simulink model "sm_car_"  (R2026b)
settings: Solver=ode23t  StopTime=100  MaxStep=0.4  AbsTol=1e-3  EnableMultiTasking=on
PreLoadFcn:
  | % Due to usability issue in Repeating Sequence block
  | warning('off','Simulink:Masking:Invalid');
  | 
  | % Eliminate unnecessary warnings in inactive variants
  | % Warnings generated only if you click through inactive variant
  | warning('off','MATLAB:nonExistentField');
  | warning('off','Simulink:Parameters:BlkParamUndefined');
PostLoadFcn:
  | set_param([bdroot '/Vehicle'],'popup_trailer','Off')
  | warning('off','sm:sli:setup:compile:LocalSolverNotSupported')
  | %sm_car_config_maneuver(bdroot,'WOT Braking');
  | sm_car_config_vehicle(bdroot,'false');
  | sm_car_config_logging(bdroot);
InitFcn:
  | sm_car_config_camera;
  | Vehicle = sm_car_vehcfg_checkConfig(Vehicle);
  | sm_car_check_tire_model(bdroot);
StartFcn:
  | tic;
StopFcn:
  | Elapsed_Sim_Time = toc;
  | % disp(['Elapsed Sim Time = ' num2str(Elapsed_Sim_Time)]);
undefined symbols (not defined in the file or in its folder): acc_theta, accel_ramp_rate, Axle1D, AxleIn, Camera, Control, Driver, Init, Maneuver, Pedal, Scene, ShaftL1, ShaftL2, ShaftR1, ShaftR2, Visual, X, xy_data_car_side, Y, Z
libraries: sm_lib x290, fl_lib x171, nesl_utility x144, simulink x60, simulink_extras x14, sdl_lib x14, SimscapeFluids_lib x7, Damper_Element x4, Tire_1x2x x4, ee_lib x3, Scene_Utilities x3, sharedTrackingLibrary x2
(part 1 of 22)
CloseFcn:
  | try,close(h1_sm_car),end
  | clear h1_sm_car
  | try,close(h2_sm_car),end
  | clear h2_sm_car
  | try,close(h3_sm_car),end
  | clear h3_sm_car
  | try,close(h4_sm_car),end
  | clear h4_sm_car
  | 
  | 
  | clear simlog_sm_car
  | clear logsout_sm_car
settings Model: SimulationMode=accelerator  Creator=smiller  LastModifiedBy=andrei
settings SolverCC: AutoInsertRateTranBlk=on  InsertRTBMode=Never (minimum delay)  MaxConsecutiveMinStep=5  MinimalZcImpactIntegration=on
settings DataIOCC: DSMLogging=off  MaxDataPoints=10000  ReturnWorkspaceOutputs=off  SaveFormat=StructureWithTime  SaveOutput=off  SignalLoggingName=logsout_sm_car
settings OptimizationCC: BlockReduction=off  BufferReuse=off  BusAssignmentInplaceUpdate=off  ExpressionFolding=off  GlobalBufferReuse=off  LocalBlockOutputs=off  OptimizeBlockIOStorage=off  OptimizeDataStoreBuffers=off  ReuseModelBlockBuffer=off  UseDivisionForNetSlopeComputation=on
settings DebuggingCC: AlgebraicLoopMsg=none  ArithmeticOperatorsInVariantConditions=warning  ParameterPrecisionLossMsg=none
settings HardwareCC: ProdHWDeviceType=Generic->32-bit x86 compatible  ProdLargestAtomicFloat=None  ProdLongLongMode=on
settings SFSimCC: CustomCodeUndefinedFunction=UseInterfaceOnly
settings RTWCC: DLArmComputeVersion=19.05
settings GRTTargetCC: TargetLangStandard=C89/C90 (ANSI)
settings SimscapeCC: SimscapeLogName=simlog_sm_car  SimscapeLogSimulationStatistics=on  SimscapeLogType=all  SimscapeOperatingPoint=ssc_op  SimscapeUseEnergyAccounting=off
settings DiagnosticsConfigSet: SimMechanicsConflictingReferenceFrames=none  SimMechanicsRigidlyBoundBlock=none  SimMechanicsUnsatisfiedHighPriorityTargets=error
settings ExplorerConfigSet: InternalSimMechanicsExplorerSettings="<ExplorerConfiguration><canonicalview>default</canonicalview><AnimationSetting><BasePlaybackSpeed>1.0</BasePlaybackSpeed><PlaybackSpeedFactor>1.0</PlaybackSpeedFactor></AnimationSetting><TilePanel><TileInfo><Tiles Columns=\"1\" Count=\"1\" Rows=\"1\"><Column Weight=\"1\"/><Row Weight=\"1\"/><Tile Height=\"1\" Width=\"1\" X=\"0\" Y=\"0\"/></Tiles></TileInfo><SceneInfo><SceneViewer><BGColor><R>1</R><G>1</G><B>1</B></BGColor><Camera><DoPerspective>on</DoPerspective><Position><X>-22.5734563329168161</X><Y>-2.56079992530625722</Y><Z>1.4393604008155032</Z></Position><Center><X>-23.2962680852000119</X><Y>-1.95845679840359432</Y><Z>1.10064823948317181</Z></Center><Up><X>-0.260205889993916473</X><Y>0.216838241661597014</Y><Z>0.940890042335224552</Z></Up><ViewLimDist>1</ViewLimDist><YLim>0.466307658154998694</YLim><XLim>0.489818968650208741</XLim></Camera></SceneViewer></SceneInfo></TilePanel><MechEditorPanel><Cameras><Camera><Id>Camera1</Id><Value><Name>Track FixO FR</Name><NativeCamera><PositionTrackingFeature>Camera_Frames.Frame_FixO_FR.R</PositionTrackingFeature><CenterTrackingFeature>Camera_Frames.Frame_FixO_FR.R</CenterTrackingFeature><UpVectorTrackingFeature>Camera_Frames.Frame_FixO_FR.R</UpVectorTrackingFeature><CenterTrackingOrigin>off</CenterTrackingOrigin><CenterTrackingDirection>+X</CenterTrackingDirection><UpVectorTrackingDirection>+Z</UpVectorTrackingDirection></NativeCamera></Value></Camera><Camera><Id>Camera2</Id><Value><Name>Track FixO Right</Name><NativeCamera><PositionTrackingFeature>Camera_Frames.Frame_FixO_Right.R</PositionTrackingFeature><CenterTrackingFeature>Camera_Frames.Transform_Camera_Ref.F</CenterTrackingFeature><UpVectorTrackingFeature>Camera_Frames.Frame_FixO_Right.R</UpVectorTrackingFeature><CenterTrackingOrigin>off</CenterTrackingOrigin><CenterTrackingDirection>+Y</CenterTrackingDirection><UpVectorTrackingDirection>+Z</UpVectorTrackingDirection></NativeCamera></Value></Camera><Camera><Id>Camera3</Id><Value><Name>Track FixO RR</Name><NativeCamera><PositionTrackingFeature>Camera_Frames.Frame_FixO_RR.R</PositionTrackingFeature><CenterTrackingFeature>Camera_Frames.Frame_FixO_RR.R</CenterTrackingFeature><UpVectorTrackingFeature>Camera_Frames.Frame_FixO_RR.R</UpVectorTrackingFeature><CenterTrackingOrigin>off</CenterTrackingOrigin><CenterTrackingDirection>+X</CenterTrackingDirection><UpVectorTrackingDirection>+Z</UpVectorTrackingDirection></NativeCamera></Value></Camera><Camera><Id>Camera4</Id><Value><Name>Track FixO RL</Name><NativeCamera><PositionTrackingFeature>Camera_Frames.Frame_FixO_RL.R</PositionTrackingFeature><CenterTrackingFeature>Camera_Frames.Frame_FixO_RL.R</CenterTrackingFeature><UpVectorTrackingFeature>Camera_Frames.Frame_FixO_RL.R</UpVectorTrackingFeature><CenterTrackingOrigin>off</CenterTrackingOrigin><CenterTrackingDirection>+X</CenterTrackingDirection><UpVectorTrackingDirection>+Z</UpVectorTrackingDirection></NativeCamera></Value></Camera><Camera><Id>Camera5</Id><Value><Name>Track FixO Left</Name><NativeCamera><PositionTrackingFeature>Camera_Frames.Frame_FixO_Left.R</PositionTrackingFeature><CenterTrackingFeature>Camera_Frames.Transform_Camera_Ref.F</CenterTrackingFeature><UpVectorTrackingFeature>Camera_Frames.Frame_FixO_Left.R</UpVectorTrackingFeature><CenterTrackingOrigin>off</CenterTrackingOrigin><CenterTrackingDirection>-Y</CenterTrackingDirection><UpVectorTrackingDirection>+Z</UpVectorTrackingDirection></NativeCamera></Value></Camera><Camera><Id>Camera6</Id><Value><Name>Track FixO FL</Name><NativeCamera><PositionTrackingFeature>Camera_Frames.Frame_FixO_FL.R</PositionTrackingFeature><CenterTrackingFeature>Camera_Frames.Frame_FixO_FL.R</CenterTrackingFeature><UpVectorTrackingFeature>Camera_Frames.Frame_FixO_FL.R</UpVectorTrackingFeature><CenterTrackingOrigin>off</CenterTrackingOrigin><CenterTrackingDirection>+X</CenterTrackingDirection><UpVectorTrackingDirection>+Z</UpVectorTrackingDirection></NativeCamera></Value></Camera><Camera><Id>Camera7</Id><Value><Name>Track FixO Top</Name><NativeCamera><PositionTrackingFeature>Camera_Frames.Frame_FixO_Top.R</PositionTrackingFeature><CenterTrackingFeature>Camera_Frames.Frame_FixO_Top.R</CenterTrackingFeature><UpVectorTrackingFeature>Camera_Frames.Frame_FixO_Top.R</UpVectorTrackingFeature><CenterTrackingOrigin>off</CenterTrackingOrigin><CenterTrackingDirection>+X</CenterTrackingDirection><UpVectorTrackingDirection>+Z</UpVectorTrackingDirection></NativeCamera></Value></Camera><Camera><Id>Camera8</Id><Value><Name>Track FixO Front</Name><NativeCamera><PositionTrackingFeature>Camera_Frames.Frame_FixO_Front.R</PositionTrackingFeature><CenterTrackingFeature>Camera_Frames.Frame_FixO_Front.R</CenterTrackingFeature><UpVectorTrackingFeature>Camera_Frames.Frame_FixO_Front.R</UpVectorTrackingFeature><CenterTrackingOrigin>off</CenterTrackingOrigin><CenterTrackingDirection>+X</CenterTrackingDirection><UpVectorTrackingDirection>+Z</UpVectorTrackingDirection></NativeCamera></Value></Camera><Camera><Id>Camera9</Id><Value><Name>Track FixO Rear</Name><NativeCamera><PositionTrackingFeature>Camera_Frames.Frame_FixO_Rear.R</PositionTrackingFeature><CenterTrackingFeature>Camera_Frames.Frame_FixO_Rear.R</CenterTrackingFeature><UpVectorTrackingFeature>Camera_Frames.Frame_FixO_Rear.R</UpVectorTrackingFeature><CenterTrackingOrigin>off</CenterTrackingOrigin><CenterTrackingDirection>+X</CenterTrackingDirection><UpVectorTrackingDirection>+Z</UpVectorTrackingDirection></NativeCamera></Value></Camera><Camera><Id>Camera10</Id><Value><Name>Track FR</Name><NativeCamera><PositionTrackingFeature>Camera_Frames.Frame_FR.R</PositionTrackingFeature><CenterTrackingFeature>Camera_Frames.Frame_FR.R</CenterTrackingFeature><UpVectorTrackingFeature>Camera_Frames.Frame_FR.R</UpVectorTrackingFeature><CenterTrackingOrigin>off</CenterTrackingOrigin><CenterTrackingDirection>+X</CenterTrackingDirection><UpVectorTrackingDirection>+Z</UpVectorTrackingDirection></NativeCamera></Value></Camera><Camera><Id>Camera11</Id><Value><Name>Track Right</Name><NativeCamera><PositionTrackingFeature>Camera_Frames.Frame_Right.R</PositionTrackingFeature><CenterTrackingFeature>Camera_Frames.Transform_Camera_Ref.F</CenterTrackingFeature><UpVectorTrackingFeature>Camera_Frames.Frame_Right.R</UpVectorTrackingFeature><CenterTrackingOrigin>off</CenterTrackingOrigin><CenterTrackingDirection>+Y</CenterTrackingDirection><UpVectorTrackingDirection>+Z</UpVectorTrackingDirection></NativeCamera></Value></Camera><Camera><Id>Camera12</Id><Value><Name>Track RR</Name><NativeCamera><PositionTrackingFeature>Camera_Frames.Frame_RR.R</PositionTrackingFeature><CenterTrackingFeature>Camera_Frames.Frame_RR.R</CenterTrackingFeature><UpVectorTrackingFeature>Camera_Frames.Frame_RR.R</UpVectorTrackingFeature><CenterTrackingOrigin>off</CenterTrackingOrigin><CenterTrackingDirection>+X</CenterTrackingDirection><UpVectorTrackingDirection>+Z</UpVectorTrackingDirection></NativeCamera></Value></Camera><Camera><Id>Camera13</Id><Value><Name>Track RL</Name><NativeCamera><PositionTrackingFeature>Camera_Frames.Frame_RL.R</PositionTrackingFeature><CenterTrackingFeature>Camera_Frames.Frame_RL.R</CenterTrackingFeature><UpVectorTrackingFeature>Camera_Frames.Frame_RL.R</UpVectorTrackingFeature><CenterTrackingOrigin>off</CenterTrackingOrigin><CenterTrackingDirection>+X</CenterTrackingDirection><UpVectorTrackingDirection>+Z</UpVectorTrackingDirection></NativeCamera></Value></Camera><Camera><Id>Camera14</Id><Value><Name>Track Left</Name><NativeCamera><PositionTrackingFeature>Camera_Frames.Frame_Left.R</PositionTrackingFeature><CenterTrackingFeature>Camera_Frames.Transform_Camera_Ref.F</CenterTrackingFeature><UpVectorTrackingFeature>Camera_Frames.Frame_Left.R</UpVectorTrackingFeature><CenterTrackingOrigin>off</CenterTrackingOrigin><CenterTrackingDirection>-Y</CenterTrackingDirection><UpVectorTrackingDirection>+Z</UpVectorTrackingDirection></NativeCamera></Value></Camera><Camera><Id>Camera15</Id><Value><Name>Track FL</Name><NativeCamera><PositionTrackingFeature>Camera_Frames.Frame_FL.R</PositionTrackingFeature><CenterTrackingFeature>Camera_Frames.Frame_FL.R</CenterTrackingFeature><UpVectorTrackingFeature>Camera_Frames.Frame_FL.R</UpVectorTrackingFeature><CenterTrackingOrigin>off</CenterTrackingOrigin><CenterTrackingDirection>+X</CenterTrackingDirection><UpVectorTrackingDirection>+Z</UpVectorTrackingDirection></NativeCamera></Value></Camera><Camera><Id>Camera16</Id><Value><Name>Track Top</Name><NativeCamera><PositionTrackingFeature>Camera_Frames.Frame_Top.R</PositionTrackingFeature><CenterTrackingFeature>Camera_Frames.Frame_Top.R</CenterTrackingFeature><UpVectorTrackingFeature>Camera_Frames.Frame_Top.R</UpVectorTrackingFeature><CenterTrackingOrigin>off</CenterTrackingOrigin><CenterTrackingDirection>+X</CenterTrackingDirection><UpVectorTrackingDirection>+Z</UpVectorTrackingDirection></NativeCamera></Value></Camera><Camera><Id>Camera17</Id><Value><Name>Track Front</Name><NativeCamera><PositionTrackingFeature>Camera_Frames.Frame_Front.R</PositionTrackingFeature><CenterTrackingFeature>Camera_Frames.Frame_Front.R</CenterTrackingFeature><UpVectorTrackingFeature>Camera_Frames.Frame_Front.R</UpVectorTrackingFeature><CenterTrackingOrigin>off</CenterTrackingOrigin><CenterTrackingDirection>+X</CenterTrackingDirection><UpVectorTrackingDirection>+Z</UpVectorTrackingDirection></NativeCamera></Value></Camera><Camera><Id>Camera18</Id><Value><Name>Track Rear</Name><NativeCamera><PositionTrackingFeature>Camera_Frames.Frame_Rear.R</PositionTrackingFeature><CenterTrackingFeature>Camera_Frames.Frame_Rear.R</CenterTrackingFeature><UpVectorTrackingFeature>Camera_Frames.Frame_Rear.R</UpVectorTrackingFeature><CenterTrackingOrigin>off</CenterTrackingOrigin><CenterTrackingDirection>+X</CenterTrackingDirection><UpVectorTrackingDirection>+Z</UpVectorTrackingDirection></NativeCamera></Value></Camera><Camera><Id>Camera19</Id><Value><Name>Track SuspF</Name><NativeCamera><PositionTrackingFeature>Camera_Frames.Frame_SuspF.R</PositionTrackingFeature><CenterTrackingFeature>Camera_Frames.Frame_SuspF.R</CenterTrackingFeature><UpVectorTrackingFeature>Camera_Frames.Frame_SuspF.R</UpVectorTrackingFeature><CenterTrackingOrigin>off</CenterTrackingOrigin><CenterTrackingDirection>+X</CenterTrackingDirection><UpVectorTrackingDirection>+Z</UpVectorTrackingDirection></NativeCamera></Value></Camera><Camera><Id>Camera20</Id><Value><Name>Track SuspR</Name><NativeCamera><PositionTrackingFeature>Camera_Frames.Frame_SuspR.R</PositionTrackingFeature><CenterTrackingFeature>Camera_Frames.Frame_SuspR.R</CenterTrackingFeature><UpVectorTrackingFeature>Camera_Frames.Frame_SuspR.R</UpVectorTrackingFeature><CenterTrackingOrigin>off</CenterTrackingOrigin><CenterTrackingDirection>+X</CenterTrackingDirection><UpVectorTrackingDirection>+Z</UpVectorTrackingDirection></NativeCamera></Value></Camera><Camera><Id>Camera21</Id><Value><Name>Track WheelFR</Name><NativeCamera><PositionTrackingFeature>Camera_Frames.Frame_Wheel_FR.R</PositionTrackingFeature><CenterTrackingFeature>Camera_Frames.Frame_Wheel_FR.R</CenterTrackingFeature><UpVectorTrackingFeature>Camera_Frames.Frame_Wheel_FR.R</UpVectorTrackingFeature><CenterTrackingOrigin>off</CenterTrackingOrigin><CenterTrackingDirection>+X</CenterTrackingDirection><UpVectorTrackingDirection>+Z</UpVectorTrackingDirection></NativeCamera></Value></Camera><Camera><Id>Camera22</Id><Value><Name>Track WheelRR</Name><NativeCamera><PositionTrackingFeature>Camera_Frames.Frame_Wheel_RR.R</PositionTrackingFeature><CenterTrackingFeature>Camera_Frames.Frame_Wheel_RR.R</CenterTrackingFeature><UpVectorTrackingFeature>Camera_Frames.Frame_Wheel_RR.R</UpVectorTrackingFeature><CenterTrackingOrigin>off</CenterTrackingOrigin><CenterTrackingDirection>+X</CenterTrackingDirection><UpVectorTrackingDirection>+Z</UpVectorTrackingDirection></NativeCamera></Value></Camera><Camera><Id>Camera23</Id><Value><Name>Track WheelRL</Name><NativeCamera><PositionTrackingFeature>Camera_Frames.Frame_Wheel_RL.R</PositionTrackingFeature><CenterTrackingFeature>Camera_Frames.Frame_Wheel_RL.R</CenterTrackingFeature><UpVectorTrackingFeature>Camera_Frames.Frame_Wheel_RL.R</UpVectorTrackingFeature><CenterTrackingOrigin>off</CenterTrackingOrigin><CenterTrackingDirection>+X</CenterTrackingDirection><UpVectorTrackingDirection>+Z</UpVectorTrackingDirection></NativeCamera></Value></Camera><Camera><Id>Camera24</Id><Value><Name>Track WheelFL</Name><NativeCamera><PositionTrackingFeature>Camera_Frames.Frame_Wheel_FL.R</PositionTrackingFeature><CenterTrackingFeature>Camera_Frames.Frame_Wheel_FL.R</CenterTrackingFeature><UpVectorTrackingFeature>Camera_Frames.Frame_Wheel_FL.R</UpVectorTrackingFeature><CenterTrackingOrigin>off</CenterTrackingOrigin><CenterTrackingDirection>+X</CenterTrackingDirection><UpVectorTrackingDirection>+Z</UpVectorTrackingDirection></NativeCamera></Value></Camera><Camera><Id>Camera25</Id><Value><Name>View Seat FL</Name><NativeCamera><PositionTrackingFeature>Camera_Frames.Frame_View_Seat_FL.R</PositionTrackingFeature><CenterTrackingFeature>Camera_Frames.Frame_View_Seat_FL.R</CenterTrackingFeature><UpVectorTrackingFeature>Camera_Frames.Frame_View_Seat_FL.R</UpVectorTrackingFeature><CenterTrackingOrigin>off</CenterTrackingOrigin><CenterTrackingDirection>+X</CenterTrackingDirection><UpVectorTrackingDirection>+Z</UpVectorTrackingDirection></NativeCamera></Value></Camera><Camera><Id>Camera26</Id><Value><Name>View Seat FR</Name><NativeCamera><PositionTrackingFeature>Camera_Frames.Frame_View_Seat_FR.R</PositionTrackingFeature><CenterTrackingFeature>Camera_Frames.Frame_View_Seat_FR.R</CenterTrackingFeature><UpVectorTrackingFeature>Camera_Frames.Frame_View_Seat_FR.R</UpVectorTrackingFeature><CenterTrackingOrigin>off</CenterTrackingOrigin><CenterTrackingDirection>+X</CenterTrackingDirection><UpVectorTrackingDirection>+Z</UpVectorTrackingDirection></NativeCamera></Value></Camera><Camera><Id>Camera27</Id><Value><Name>View Susp FR</Name><NativeCamera><PositionTrackingFeature>Camera_Frames.Frame_View_Susp_FR.R</PositionTrackingFeature><CenterTrackingFeature>Camera_Frames.Frame_View_Susp_FR.R</CenterTrackingFeature><UpVectorTrackingFeature>Camera_Frames.Frame_View_Susp_FR.R</UpVectorTrackingFeature><CenterTrackingOrigin>off</CenterTrackingOrigin><CenterTrackingDirection>+X</CenterTrackingDirection><UpVectorTrackingDirection>+Z</UpVectorTrackingDirection></NativeCamera></Value></Camera><Camera><Id>Camera28</Id><Value><Name>View Susp RR</Name><NativeCamera><PositionTrackingFeature>Camera_Frames.Frame_View_Susp_RR.R</PositionTrackingFeature><CenterTrackingFeature>Camera_Frames.Frame_View_Susp_RR.R</CenterTrackingFeature><UpVectorTrackingFeature>Camera_Frames.Frame_View_Susp_RR.R</UpVectorTrackingFeature><CenterTrackingOrigin>off</CenterTrackingOrigin><CenterTrackingDirection>+X</CenterTrackingDirection><UpVectorTrackingDirection>+Z</UpVectorTrackingDirection></NativeCamera></Value></Camera><Camera><Id>Camera29</Id><Value><Name>View Susp RL</Name><NativeCamera><PositionTrackingFeature>Camera_Frames.Frame_View_Susp_RL.R</PositionTrackingFeature><CenterTrackingFeature>Camera_Frames.Frame_View_Susp_RL.R</CenterTrackingFeature><UpVectorTrackingFeature>Camera_Frames.Frame_View_Susp_RL.R</UpVectorTrackingFeature><CenterTrackingOrigin>off</CenterTrackingOrigin><CenterTrackingDirection>+X</CenterTrackingDirection><UpVectorTrackingDirection>+Z</UpVectorTrackingDirection></NativeCamera></Value></Camera><Camera><Id>Camera30</Id><Value><Name>View Susp FL</Name><NativeCamera><PositionTrackingFeature>Camera_Frames.Frame_View_Susp_FL.R</PositionTrackingFeature><CenterTrackingFeature>Camera_Frames.Frame_View_Susp_FL.R</CenterTrackingFeature><UpVectorTrackingFeature>Camera_Frames.Frame_View_Susp_FL.R</UpVectorTrackingFeature><CenterTrackingOrigin>off</CenterTrackingOrigin><CenterTrackingDirection>+X</CenterTrackingDirection><UpVectorTrackingDirection>+Z</UpVectorTrackingDirection></NativeCamera></Value></Camera><Camera><Id>Camera31</Id><Value><Name>Dolly Camera</Name><NativeCamera><PositionTrackingFeature>Camera_Frames.Frame_Dolly.R</PositionTrackingFeature><CenterTrackingFeature>Camera_Frames.Frame_Dolly.R</CenterTrackingFeature><UpVectorTrackingFeature>Camera_Frames.Frame_Dolly.R</UpVectorTrackingFeature><CenterTrackingOrigin>off</CenterTrackingOrigin><CenterTrackingDirection>+X</CenterTrackingDirection><UpVectorTrackingDirection>+Z</UpVectorTrackingDirection></NativeCamera></Value></Camera><Camera><Id>Camera32</Id><Value><Name>Track Dolly Camera</Name><NativeCamera><PositionTrackingFeature>Camera_Frames.Frame_Dolly.R</PositionTrackingFeature><CenterTrackingFeature>Camera_Frames.Transform_Camera_Ref.F</CenterTrackingFeature><UpVectorTrackingFeature>Camera_Frames.World_Frame.W</UpVectorTrackingFeature><CenterTrackingOrigin>on</CenterTrackingOrigin><UpVectorTrackingDirection>+Z</UpVectorTrackingDirection></NativeCamera></Value></Camera></Cameras><GfxPanelCameraMap><MapElement CameraMLId=\"Camera1\" GfxPanelIndex=\"0\"/></GfxPanelCameraMap><VideoCreator><PlaybackSpeedRatio>1.0</PlaybackSpeedRatio><FrameRate>30</FrameRate><VideoFormat>MPEG-4</VideoFormat><FrameSize>[800 450]</FrameSize></VideoCreator></MechEditorPanel></ExplorerConfiguration>"

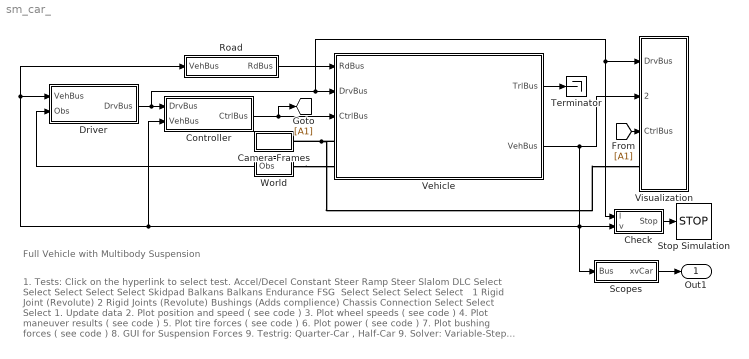
== system sm_car_ ==
  note: Full Vehicle with Multibody Suspension
  note: 1. Tests: Click on the hyperlink to select test.
      | Accel/Decel
      | Constant Steer
      | Ramp Steer
      | Slalom
      | DLC
      |
      | Select
      | Select
      | Select
      | Select
      | Select
      |
      | Skidpad
      | Balkans
      | Balkans Endurance
      | FSG
      | ​
      |
      | Select
      | Select
      | Select
      | Select
      | ​
      |
      | ​
      | 1 Rigid Joint
      | (Revolute)
      | 2 Rigid Joints
      | (Revolute)
      | Bushings
      | (Adds complience)
      |
      | Chassis Connection
      | Select
      | Select
      | Select
      |
      | 1. Update data
      | 2. Plot position and speed ( see code )
      | 3. Plot wheel speeds ( see code )
      | 4. Plot maneuver results ( see code )
      | 5. Plot tire forces ( see code )
      | 6. Plot power ( see code )
      | 7. Plot bushing forces ( see code )
      | 8. GUI for Suspension Forces
      | 9. Testrig: Quarter-Car , Half-Car
      |
      | 9. Solver: Variable-Step , Fixed Step ( see code )
      | 10. Explore simulation results using sscexplore
      | 11. Learn more about this model.
  Camera Frames : Subsystem  mask(Camera Frame Definitions){Camera=Camera, popup_dolly_camera=Off}
      mask prompts: popup_dolly_camera "Dolly Camera"
      mask help: Defines set of camera frames surrounding vehicle. Frames are used to define visualization viewpoints for animation of simulation results.
      mask init:
      | set_param([gcb '/Dolly Camera'],'LabelModeActiveChoice',get_param(gcb,'popup_dolly_camera'));
      mask TypeOptions popup_dolly_camera: Off | XYZ
      mask Display: disp('Cam')
  Check : Subsystem  mask(Stop Conditions){stop_speed=0.1, start_check_time=5, max_speed=0.4, start_check_time_max_speed=20000, lat_dev_threshold=4, start_check_time_ld=4, End_Lap=0.2, start_check_end_lap=20000, Final_lap=1, Time_Lap_Final=10000, max_dist_threshold=Maneuver.xMax.Value, start_check_time_max_dist=2}
      mask help: Check conditions of vehicle to determine if simulation should stop. Conditions can include speed, position, or end of lap. Set time to start check to very high values to prevent condition from stopping simulation.
      mask TypeOptions stop_speed: Stop Threshold/Value
      mask TypeOptions start_check_time: Start Checking/Time
      mask TypeOptions max_speed: Max Speed Threshold/Value
      mask TypeOptions start_check_time_max_speed: Start Checking Max Speed/Time
      mask TypeOptions lat_dev_threshold: Lateral Deviation Threshold/Value
      mask TypeOptions start_check_time_ld: Start Checking Lat Dev/Time
      mask TypeOptions End_Lap: End Lap/Value
      mask TypeOptions start_check_end_lap: Start Checking End Lap/Time
      mask TypeOptions Final_lap: End Laps/Value
      mask TypeOptions Time_Lap_Final: Start Checking Final Lap/Time
      mask TypeOptions max_dist_threshold: End Distance/Value
      mask TypeOptions start_check_time_max_dist: Start Checking End Distance/Time
      mask DialogControl text_quantity Prompt: Quantity
      mask DialogControl text_start_check Prompt: Start Check (sec)
      mask DialogControl text_final_speed Prompt: Final Speed (m/s)
      mask DialogControl text_max_speed Prompt: Max Speed (m/s)
      mask DialogControl text_max_lat_dev Prompt: Max Lateral Offset (m)
      mask DialogControl text_end_lap Prompt: End Lap
      mask DialogControl text_final_lap Prompt: Final Lap
      mask DialogControl text_max_distance Prompt: Max Distance
  Controller : Subsystem  Variant=on  VariantControlMode=label  VariantControl=Variant1  LabelModeActiveChoice=Default  mask(Control){popup_control=Default, popup_brake_control=Pedal}
      mask prompts: popup_control "Control"; popup_brake_control "Brake Control"
      mask help: Models vehicle controller behavior. Takes commands from driver and produces inputs for vehicle systems including braking, steering, and powertrain.
      mask init:
      | temp_ctrlMode = get_param(gcb,'popup_control');
      | if(strcmp(temp_ctrlMode,'Default'))
      |     set_param(gcb,'LabelModeActiveChoice','Default');
      |     set_param([gcb '/Default'],'popup_brake_control',...
      |         get_param(gcb,'popup_brake_control'))
      | elseif(strcmp(temp_ctrlMode,'Fuel Cell 1 Motor'))
      |     set_param(gcb,'LabelModeActiveChoice','FuelCell1Motor');
      | elseif(strcmp(temp_ctrlMode,'Battery 2 Motor'))
      |     set_param(gcb,'LabelModeActiveChoice','Battery2Motor');
      | elseif(strcmp(temp_ctrlMode,'Torque Vector 4 Motor'))
      |     set_param(gcb,'LabelModeActiveChoice','TrqVec_4Motor');
      |     set_param([gcb '/TrqVec 4Motor'],'popup_brake_control',...
      |         get_param(gcb,'popup_brake_control'))
      | elseif(strcmp(temp_ctrlMode,'TrqVecARTTU'))
      |         set_param(gcb,'LabelModeActiveChoice','TrqVecARTTU');
      | elseif(strcmp(temp_ctrlMode,'FLC_DYC'))
      |         set_param(gcb,'LabelModeActiveChoice','FLC_DYC');
      | elseif(strcmp(temp_ctrlMode,'FLC_DYC_V2'))
      |         set_param(gcb,'LabelModeActiveChoice','FLC_DYC_V2');
      | elseif(strcmp(temp_ctrlMode,'FLC_DYC_V3'))
      |         set_param(gcb,'LabelModeActiveChoice','FLC_DYC_V3');
      | elseif(strcmp(temp_ctrlMode,'Slip_Ctrl'))
      |         set_param(gcb,'LabelModeActiveChoice','Slip_Ctrl');
      | elseif(strcmp(temp_ctrlMode,'FeedF_Ctrl'))
      |         set_param(gcb,'LabelModeActiveChoice','FeedF_Ctrl');
      | elseif(strcmp(temp_ctrlMode,'Slip_Ctrl_V2'))
      |         set_param(gcb,'LabelModeActiveChoice','Slip_Ctrl_V2');
      | end
      settings: AttributesFormatString=%<popup_control>
      mask TypeOptions popup_control: Default | FLC_DYC_V3 | Slip_Ctrl_V2 | FeedF_Ctrl | Slip_Ctrl | FLC_DYC | FLC_DYC_V2 | NoIMU | Torque Vector 4 Motor
      mask Callback popup_control:
      | maskObj = get_param(gcb,'MaskObject');
      | pbc_h = maskObj.getParameter('popup_brake_control');
      | control_value = get_param(gcb,'popup_control');
      | if(strcmp(control_value,'Default') || strcmp(control_value,'Torque Vector 4 Motor') || strcmp(control_value,'TrqVecARTTU'))
      |     pbc_h.Visible = 'on';
      | else
      |     pbc_h.Visible = 'off';
      | end
      mask TypeOptions popup_brake_control: Pedal
      mask Display: disp(' ');
  Driver : Subsystem  AncestorBlock=Driver/Driver  Variant=on  VariantControlMode=label  VariantControl=Variant1  LabelModeActiveChoice=Closed_Loop1  mask(Driver){popup_driver_type=Closed Loop1}
      mask prompts: popup_driver_type "Driver"
      mask help: Models driver behavior. Open loop driver specifies positions of accelerator, brake pedal, and steering wheel. Closed loop driver compares current vehicle pose (x, y, theta) and current vehicle speed with target position and speed.
      mask init:
      | set_param(gcb,'LabelModeActiveChoice',strrep(get_param(gcb,'popup_driver_type'),' ','_'));
      settings: AttributesFormatString=%<popup_driver_type>
      mask TypeOptions popup_driver_type: Closed Loop | Closed Loop1 | Open Loop
      mask Display: disp(' ')
  Road : Subsystem
  Scopes : Subsystem
  Stop Simulation : Stop
  Terminator : Terminator
  Vehicle : Subsystem  mask(Vehicle with Optional Trailer){popup_trailer=Off}
      mask prompts: popup_trailer "Trailer"
      mask help: Models a two-axle vehicle with optional single axle trailer. Configuration and fidelity level of suspension, powertrain, tires, and more set by fields in Vehicle data structure.
      mask init:
      | if(strcmp(get_param(gcb,'popup_trailer'),'On'))
      |     set_param([gcb '/Trailer'],'LabelModeActiveChoice','Trailer');
      | else
      |     set_param([gcb '/Trailer'],'LabelModeActiveChoice','None');
      | end
      mask TypeOptions popup_trailer: On | Off
      mask Display:
      | % Assemble image from BodyGeometry.class
      | % (active choice from Body Geometry subsystem)
      | 
      | temp_trl_bg_class = 'none';
      | if(strcmp(get_param(gcb,'popup_trailer'),'On'))
      |     temp_trl_bg_class = lower(get_param([gcb '/Trailer/Trailer/Chassis/Body/Body Geometry'],'LabelModeActiveChoice'));
      | end
      | temp_veh_bg_class = lower(get_param([gcb '/Vehicle/Chassis/Body/Body Geometry'],'LabelModeActiveChoice'));
      | 
      | imagestr = (['sm_car_vehicle_' temp_veh_bg_class '_' temp_trl_bg_class '.png']);
      | 
      | % If image does not exist, use default image
      | % Changes based on trailer popup
      | if(~exist(imagestr))
      |     if(strcmp(get_param(gcb,'popup_trailer'),'On'))
      |         temp_trl_bg_class = 'default';
      |     else
      |         temp_trl_bg_class = 'none';
      |     end
      |     imagestr = ['sm_car_vehicle_axle2_default_' temp_trl_bg_class '.png'];
      | end
      | 
      | image(imagestr);
  Visualization : Subsystem  mask(Unreal Visualization){unreal_onoff=Off, torque_bars_onoff=Off}
      mask prompts: unreal_onoff "Unreal Animation"; torque_bars_onoff "Rear motor torque bars"
      mask help: Optionally enable Unreal visualization of vehicle motion and scene.
      mask init:
      | set_param([gcb '/Unreal'],'popup_animation',get_param(gcb,'unreal_onoff'));
      | torque_bar_enable = double(strcmp(get_param(gcb,'torque_bars_onoff'),'On'));
      | torque_bar_opacity_scale = torque_bar_enable;
      | torque_bar_block = [gcb '/Mechanics Explorer Torque Bars'];
      | if getSimulinkBlockHandle(torque_bar_block) >= 0
      |     if torque_bar_enable
      |         set_param(torque_bar_block,'Commented','off');
      |     else
      |         set_param(torque_bar_block,'Commented','on');
      |     end
      | end
      mask TypeOptions unreal_onoff: Off
      mask TypeOptions torque_bars_onoff: Off | On
      mask Callback torque_bars_onoff:
      | torque_bar_block = [gcb '/Mechanics Explorer Torque Bars'];
      | if getSimulinkBlockHandle(torque_bar_block) >= 0
      |     if strcmp(get_param(gcb,'torque_bars_onoff'),'On')
      |         set_param(torque_bar_block,'Commented','off');
      |     else
      |         set_param(torque_bar_block,'Commented','on');
      |     end
      | end
  World : Subsystem  mask(Environment){UseLocalSolver=off, LocalSolverChoice=Backward Euler, LocalSolverSampleTime=0.002, DoFixedCost=off, MaxNonlinIter=2, popup_scene=Skidpad, popup_gravity=Constant, GravityVector=[0 0 -9.80665]}
      mask prompts: UseLocalSolver "Use Local Solver"; LocalSolverChoice "Solver Type:"; LocalSolverSampleTime "Sample time"; DoFixedCost "Use fixed-cost"; MaxNonlinIter "Number of iterations"; popup_scene "Scene"; popup_gravity "Gravity Model"; GravityVector "Gravity Vector [x y z] (m/s^2)"
      mask help: World frame, driving surface, gravity, and solver settings.
      mask init:
      | if(LocalSolverChoice == 1)
      |     solverChoice = 'NE_BACKWARD_EULER_ADVANCER';
      | elseif(LocalSolverChoice == 2)
      |     solverChoice = 'NE_TRAPEZOIDAL_ADVANCER';
      | elseif(LocalSolverChoice == 3)
      |     solverChoice = 'NE_PARTITIONING_ADVANCER';
      | end
      | set_param([gcb '/Solver Configuration'],'LocalSolverChoice',solverChoice)
      | 
      | tempblkscenename = strrep(get_param(gcb,'popup_scene'),' ','_');
      | set_param([gcb '/Scene'],'LabelModeActiveChoice',tempblkscenename);
      | gravityModel = get_param(gcb,'popup_gravity');
      | if(strcmpi(gravityModel,'constant'))
      |     set_param([gcb '/Mechanism Configuration'],'LabelModeActiveChoice','ConstantGravity');
      | elseif(strcmpi(gravityModel,'ramp x and y components'))
      |     set_param([gcb '/Mechanism Configuration'],'LabelModeActiveChoice','VariableGravityXY');
      | end
      | clear tempblkscenename
      settings: AttributesFormatString=|
      | %<popup_scene>
      | Local Solver: %<UseLocalSolver>
      mask TypeOptions UseLocalSolver:
      | Solver
      | Configuration/UseLocalSolver
      mask Callback UseLocalSolver:
      | maskObj = Simulink.Mask.get(gcb);
      | 
      | samTM_h = maskObj.getParameter('LocalSolverSampleTime');
      | slvCH_h = maskObj.getParameter('LocalSolverChoice');
      | fixCT_h = maskObj.getParameter('DoFixedCost');
      | 
      | temp_useLSstate = get_param(gcb,'UseLocalSolver');
      | samTM_h.Enabled = temp_useLSstate;
      | slvCH_h.Enabled = temp_useLSstate;
      | fixCT_h.Enabled = temp_useLSstate;
      | 
      | clear maskObj
      | clear samTM_h slvCH_h fixCT_h
      | clear temp_useLSstate
      mask TypeOptions LocalSolverChoice: Backward Euler | Trapezoidal Rule | Partitioning
      mask TypeOptions LocalSolverSampleTime:
      | Solver
      | Configuration/LocalSolverSampleTime
      mask TypeOptions DoFixedCost:
      | Solver
      | Configuration/DoFixedCost
      mask Callback DoFixedCost:
      | maskObj = Simulink.Mask.get(gcb);
      | 
      | numIT_h = maskObj.getParameter('MaxNonlinIter');
      | 
      | temp_doFixCoststate = get_param(gcb,'DoFixedCost');
      | numIT_h.Enabled = temp_doFixCoststate;
      | 
      | clear maskObj numIT_h temp_doFixCoststate
      mask TypeOptions MaxNonlinIter:
      | Solver
      | Configuration/MaxNonlinIter
      mask TypeOptions popup_scene: CRG Hockenheim | CRG Germania | CRG Germania F | CRG Balkans End | CRG Balkans End F | Slalom | CRG Dej Wide | CRG Dej Wide F | CRG Balkans | CRG Balkans F | Double Lane Change | Double Lane Change ISO3888 | CRG Hockenheim F | Plane Grid | Skidpad
      mask TypeOptions popup_gravity: Constant | Ramp x and y components
      mask Display: disp('Wld')
  Out1 : Outport  VectorParamsAs1DForOutWhenUnconnected=off
  wires:
  Check/1(Stop) -> Stop Simulation/1
  Scopes/1(xvCar) -> Out1/1
  Driver/1(" DrvBus") -> Controller/1("DrvBus "), Check/1(l), Visualization/1(DrvBus), Vehicle/2(DrvBus)
  Vehicle/2(VehBus) -> Check/2(v), Scopes/1(Bus), Controller/2("VehBus "), Road/1(VehBus), Driver/1("VehBus "), Visualization/2(VehBus)
  Road/1(RdBus) -> Vehicle/1(RdBus)
  Controller/1(" CtrlBus") -> Vehicle/3(CtrlBus), [A1]
  Vehicle/1(TrlBus) -> Terminator/1
  World/1(Obs) -> Driver/2(Obs)
  [A1] -> Visualization/3(CtrlBus)
  connections:
  Vehicle/LConn1 -- Camera Frames/RConn1 -- Visualization/LConn1
  World/LConn1 -- Vehicle/LConn2
